simulink model "XFLUID02_reference"  (R2025a)
settings: Solver=ode23t  StartTime=0  StopTime=1.5  MaxStep=0.001  RelTol=1e-3  EnableMultiTasking=on
model workspace (MAT data in the model file):
  TRP_Par : object (value not decoded)
  fault_cylinder = 2
  inlet_area_factor = 1
  output_pressure_bar = 7
  pOutMeas_data = [7; 7]
  pOutMeas_time = [0; 1.5]
  pOut_Init_WKSP = 7
  pump_speed_rpm = 958
  seal_leak_fraction = 0
  speed_step_fraction = 0.08
  speed_step_time = 0.72
symbols that are objects in the model workspace (value not decoded): TRP_Par
undefined symbols (not defined in the file): Plunger, sm_pump_triplex_lib, smiData, X, Y, Z
libraries: sm_lib x133, fl_lib x62, nesl_utility x24, SimscapeFluids_lib x15, simulink x10, ee_lib x2
(part 2 of 7)

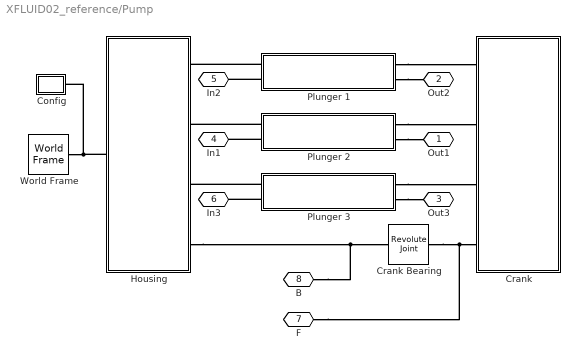
== system XFLUID02_reference/Pump ==
  Config : Subsystem
  Crank : Subsystem  mask(Crankshaft){shaft_len=shaft_len_P, shaft_rad=shaft_rad_P, web_rad=web_rad_P, web_len=web_len_P, motor_shaft_rad=motor_shaft_rad_P, motor_shaft_len=motor_shaft_len_P, shaft_pos=shaft_pos_P, crank_rho=crank_rho_P, motor_shaft_clr=motor_shaft_clr_P, crank_clr=crank_clr_P, crank_opc=crank_opc_P}
      mask prompts: shaft_pos "Crankpin Axis Offset (m)"; crank_rho "Density (kg/m^3)"; motor_shaft_clr "Motor Shaft Color [RGB]"; crank_clr "Crank Color [RGB]"; crank_opc "Opacity (0-1)"
      mask help: Models pump crankshaft with three crankpins, each offset by 120 degrees from the crankshaft axis.
      mask DialogControl text_radius Prompt: Radius (m)
      mask DialogControl text_length Prompt: Length (m)
      mask DialogControl text_crankpin Prompt: Crankpin
      mask DialogControl text_web Prompt: Web
      mask DialogControl text_motor_shaft Prompt: Motor Shaft
      mask DialogControl cont_crank_vis Prompt: Crankshaft Visualization
      mask Display: image('sm_pump_triplex_Crank_IMAGE.png');
  Crank Bearing : sm_lib/Joints/Revolute Joint  JointMode=Normal  CompositeWrenchDir=FollowerOnBase  CompositeWrenchFrame=BaseFrame  SenseConstraintForce=off  SenseConstraintTorque=off  SenseTotalForce=off  SenseTotalTorque=off  PositionTargetSpecify=off  PositionTargetPriority=High  PositionTargetValue=0  PositionTargetValueUnits=deg  VelocityTargetSpecify=off  VelocityTargetPriority=High  VelocityTargetValue=0  VelocityTargetValueUnits=deg/s  EquilibriumPosition=0  EquilibriumPositionUnits=deg  SpringStiffness=0  SpringStiffnessUnits=N*m/deg  DampingCoefficient=bearing_visc_frict  DampingCoefficientUnits=N*m/(deg/s)  LowerLimitSpecify=off  LowerLimitBound=-90  LowerLimitBoundUnits=deg  LowerLimitStiffness=1e4  LowerLimitStiffnessUnits=N*m/deg  LowerLimitDamping=10  LowerLimitDampingUnits=N*m/(deg/s)  LowerLimitTransitionRegionWidth=0.1  LowerLimitTransitionRegionWidthUnits=deg  UpperLimitSpecify=off  UpperLimitBound=90  UpperLimitBoundUnits=deg  UpperLimitStiffness=1e4  UpperLimitStiffnessUnits=N*m/deg  UpperLimitDamping=10  UpperLimitDampingUnits=N*m/(deg/s)  UpperLimitTransitionRegionWidth=0.1  UpperLimitTransitionRegionWidthUnits=deg  TorqueActuationMode=NoTorque  MotionActuationMode=ComputedMotion  SensePosition=off  SenseVelocity=off  SenseAcceleration=off  SenseTorqueForce=off  SenseLowerLimitTorqueForce=off  SenseUpperLimitTorqueForce=off
  Housing : Subsystem
      mask Display: image('sm_pump_triplex_Housing_IMAGE.png');
  Plunger 1 : Subsystem  AncestorBlock=sm_pump_triplex_lib/Plunger  mask(Hydraulic Plunger){cyl_gap=cyl_gap_P, cyl_rad_out=cyl_rad_out_P, cyl_len=cyl_len_P, cyl_stroke=cyl_stroke_P, cyl_rad_in=0, cyl_xc_rev=0, cyl_frict_brkway_frc=cyl_frict_brkway_frc_P, cyl_frict_brkway_vel=cyl_frict_brkway_vel_P, cyl_frict_col_frc=cyl_frict_col_frc_P, cyl_frict_visc_coef=cyl_frict_visc_coef_P, cyl_rho=cyl_rho_P, cyl_clr=cyl_clr_P, cyl_opc=cyl_opc_P, plgB_len=plgB_len_P, plgB_rad=plgB_rad_P, stem_len=stem_len_P, stem_rad=stem_rad_P, pin_len=pin_len_P, pin_rad=pin_rad_P, cup_rad_out=cup_rad_out_P, cup_thk=cup_thk_P, cup_len=cup_len_P, cup_pinOffset=cup_pinOffset_P, cup_rad_in=0, plg_rho=plg_rho_P, plg_clr=plg_clr_P, plg_opc=plg_opc_P, conrod_len=conrod_len_P, conrod_web_widP=conrod_web_widP_P, conrod_web_widC=conrod_web_widC_P, conrod_web_offC=0, conrod_web_offP=0, conrod_web_len=0, conrod_web_xc=0, conrod_ringC_wid=conrod_ringC_wid_P, conrod_ringP_wid=conrod_ringP_wid_P, crank_shaft_rad=crank_shaft_rad_P, conrod_ringC_or=0, conrod_ringP_or=0, conrod_ringC_xc_rev=0, conrod_ringP_xc_rev=0, conrod_thk=conrod_thk_P, conrod_rho=conrod_rho_P, conrod_clr=conrod_clr_P, conrod_opc=conrod_opc_P, chkv_in_maxA=chkv_in_maxA_P, chkv_out_maxA=chkv_out_maxA_P, chkv_press_set_popup=Set in Mask, chkv_in_crkP=chkv_in_crkP_P, chkv_out_crkP=chkv_out_crkP_P, chkv_in_maxOpenP=chkv_in_maxOpenP_P, chkv_out_maxOpenP=chkv_out_maxOpenP_P, chkv_vis_popup=Off, chkv_vis_rad_in=chkv_vis_rad_in_P, chkv_vis_rad_out=chkv_vis_rad_out_P, chkv_vis_clr_in=chkv_vis_clr_in_P, chkv_vis_clr_out=chkv_vis_clr_out_P, leak_cyl_popup=On, leak_cyl_area=1e-12+(fault_cylinder==1)*seal_leak_fraction*TRP_Par.Check_Valve.In.Max_Area, block_in_popup=On, block_in_factor=min(0.999,1-(fault_cylinder==1)*(1-inlet_area_factor)), seal_leak_vis_len=seal_leak_vis_len_P, seal_leak_vis_rad=seal_leak_vis_rad_P, seal_leak_vis_clr=seal_leak_vis_clr_P, seal_leak_vis_opc=0, inlet_obstr_len=inlet_obstr_len_P, inlet_obstr_rad=inlet_obstr_rad_P, inlet_obstr_xc_rev=0, inlet_obstr_clr=inlet_obstr_clr_P, inlet_obstr_opc=1}
      mask prompts: cyl_gap "Gap (m)"; cyl_rad_out "Outer radius (m)"; cyl_len "Length (m)"; cyl_stroke "Stroke (m)"; cyl_rad_in "Inner radius (m)"; cyl_xc_rev "Revolution Cross Section (m)"; cyl_frict_brkway_frc "Breakaway Friction Force (N)"; cyl_frict_brkway_vel "Breakaway Friction Velocity (m/s)"; cyl_frict_col_frc "Coulomb Friction Force (N)"; cyl_frict_visc_coef "Viscous Friction Coeff (N/(m/s))"; cyl_rho "Density (kg/m^3)"; cyl_clr "Color [RGB]"; cyl_opc "Opacity (0-1)"; cup_rad_out "Outer Radius (m)"; cup_thk "Wall Thickness (m)"; cup_len "Length(m)"; cup_pinOffset "Pin Offset (m)"; cup_rad_in "Inner Radius (m)"; plg_rho "Density (kg/m^3)"; plg_clr "Color [RGB]"; plg_opc "Opacity (0-1)"; conrod_len "Length, center-center (m)"; conrod_web_widP "Width, pin end (m)"; conrod_web_widC "Width, crank end (m)"; conrod_web_offC "Offset to shaft center (m)"; conrod_web_offP "Offset to pin center (m)"; conrod_web_len "Length web (m)"; conrod_web_xc "Extrusion cross section (m)"; conrod_ringC_wid "Crank Ring Width (m)"; conrod_ringP_wid "Pin Ring Width (m)"; crank_shaft_rad "Crank Shaft Radius (m)"; conrod_ringC_or "Outer Radius, Crank Ring"; conrod_ringP_or "Inner Radius, Pin Ring"; conrod_ringC_xc_rev "Crank Ring Cross Section (m)"; conrod_ringP_xc_rev "Pin Ring Cross Section (m)"; conrod_thk "Thickness (m)"; conrod_rho "Density (kg/m^3)"; conrod_clr "Color [RGB]"; conrod_opc "Opacity (0-1)"; chkv_press_set_popup "Pressure Settings"; chkv_vis_popup "Valve Visualization"; leak_cyl_popup "Seal Leak"; leak_cyl_area "Leak Area (m^2)"; block_in_popup "Blocked Inlet"; block_in_factor "Area Factor (0-1)"; seal_leak_vis_len "Length (m)"; seal_leak_vis_rad "Radius (m)"; seal_leak_vis_clr "Color [RGB]"; seal_leak_vis_opc "Opacity (0-1)"; inlet_obstr_len "Length (m)"; inlet_obstr_rad "Radius (m)"; inlet_obstr_xc_rev "Cross Section (m)"; inlet_obstr_clr "Color [RGB]"; inlet_obstr_opc "Opacity (0-1)"
      mask help: Models a single hydraulic plunger with hydraulic chamber. Two check valves control flow into and out of the hydraulic chamber. Degraded behavior can be modeled by enabling seal leakage and blocked inlet on the Faults tab. When "On, Run Time" is selected, MATLAB workspace variables set the parameters so that they can be tuned using Fast Restart.
      mask init:
      | % -- Configure submodels
      | % Fault: Seal Leak
      | if(leak_cyl_popup==1)
      |     set_param([gcb '/Seal Leak'],'OverrideUsingVariant','Off');
      |     seal_leak_vis_opc = 0;
      | elseif(leak_cyl_popup==2)
      |     set_param([gcb '/Seal Leak'],'OverrideUsingVariant','On');
      |     seal_leak_vis_opc = 1;
      | elseif(leak_cyl_popup==3)
      |     set_param([gcb '/Seal Leak'],'OverrideUsingVariant','Tune');
      |     seal_leak_vis_opc = 1;
      | end
      | 
      | % Fault: Blocked Inlet
      | inlet_obstr_xc_rev = [...
      |     inlet_obstr_rad                  -inlet_obstr_len/2;
      |     inlet_obstr_rad                   inlet_obstr_len/2;
      |     inlet_obstr_rad*block_in_factor   inlet_obstr_len/2;
      |     inlet_obstr_rad*block_in_factor  -inlet_obstr_len/2];
      | if(block_in_popup==1)
      |     set_param([gcb '/Check Valve Inlet'],...
      |         'area_max','chkv_in_maxA',...
      |         'area_max_conf','compiletime',...
      |         'BackgroundColor','[1 1 1]');
      |     inlet_obstr_opc = 0;
      | elseif(block_in_popup==2)
      |     set_param([gcb '/Check Valve Inlet'],...
      |         'area_max','chkv_in_maxA*block_in_factor',...
      |         'area_max_conf','compiletime',...
      |         'BackgroundColor','[1 0.9 0.9]');
      |     inlet_obstr_opc = 1;
      | elseif(block_in_popup==3)
      |     set_param([gcb '/Check Valve Inlet'],...
      |         'area_max','chkv_in_maxA_WKSP*block_in_factor_WKSP',...
      |         'area_max_conf','runtime',...
      |         'BackgroundColor','[1 0.9 0.9]');
      |     inlet_obstr_opc = 1;
      | end
      | 
      | % Parameter tuning: Check valve pressure settings
      | 
      | if(chkv_press_set_popup==1)
      |     set_param([gcb '/Check Valve Inlet'],...
      |         'p_crack_differential','chkv_in_crkP',...
      |         'p_crack_differential_conf','compiletime',...
      |         'press_max_differential','chkv_in_maxOpenP',...
      |         'press_max_differential_conf','compiletime');
      |     set_param([gcb '/Check Valve Outlet'],...
      |         'p_crack_differential','chkv_out_crkP',...
      |         'p_crack_differential_conf','compiletime',...
      |         'press_max_differential','chkv_out_maxOpenP',...
      |         'press_max_differential_conf','compiletime');
      | elseif(chkv_press_set_popup==2)
      |     set_param([gcb '/Check Valve Inlet'],...
      |         'p_crack_differential','chkv_all_crkP_WKSP',...
      |         'p_crack_differential_conf','runtime',...
      |         'press_max_differential','chkv_all_maxOpenP_WKSP',...
      |         'press_max_differential_conf','runtime');
      |     set_param([gcb '/Check Valve Outlet'],...
      |         'p_crack_differential','chkv_all_crkP_WKSP',...
      |         'p_crack_differential_conf','runtime',...
      |         'press_max_differential','chkv_all_maxOpenP_WKSP',...
      |         'press_max_differential_conf','runtime');
      | end
      | 
      | % Turn on/off visualization
      | if(chkv_vis_popup==1)
      |     set_param([gcb '/Valve Visual'],'OverrideUsingVariant','Off');
      | elseif(chkv_vis_popup==2)
      |     set_param([gcb '/Valve Visual'],'OverrideUsingVariant','On');
      | end
      | 
      | % -- Calculate derived parameters
      | % Cylinder: derived dimensions
      | cyl_rad_in  = plgB_rad + cyl_gap;
      | 
      | % Cylinder: cross-section for rev
      | cyl_xc_rev = [...
      |     cyl_rad_out  -cyl_len/2
      |     cyl_rad_out   cyl_len/2
      |     cyl_rad_in    cyl_len/2
      |     cyl_rad_in   -cyl_len/2];
      | 
      | % Stem Cup: cross-section for rev
      | cup_rad_in = cup_rad_out-cup_thk;
      | cup_xc_rev = [...
      |     cup_rad_out  -cup_len/2
      |     cup_rad_out   cup_len/2
      |     cup_rad_in    cup_len/2
      |     cup_rad_in   -cup_len/2];
      | 
      | % Connecting Rod, Crank Ring: cross-section for rev
      | conrod_ringC_or = crank_shaft_rad + conrod_ringC_wid;
      | conrod_ringC_xc_rev = [...
      |     conrod_ringC_or -conrod_thk/2*1.005;
      |     conrod_ringC_or  conrod_thk/2*1.005;
      |     crank_shaft_rad  conrod_thk/2*1.005;
      |     crank_shaft_rad -conrod_thk/2*1.005];
      | 
      | % Connecting Rod, Pin ring: cross-section for rev
      | conrod_ringP_or = pin_rad + conrod_ringP_wid;
      | conrod_ringP_xc_rev = [...
      |     conrod_ringP_or -conrod_thk/2*1.005;
      |     conrod_ringP_or  conrod_thk/2*1.005;
      |     pin_rad          conrod_thk/2*1.005;
      |     pin_rad         -conrod_thk/2*1.005];
      | 
      | % Connecting Rod, Web: cross-section for extrusion
      | conrod_web_offC = crank_shaft_rad + conrod_ringC_wid/2;
      | conrod_web_offP = pin_rad         + conrod_ringP_wid/2;
      | conrod_web_len  = conrod_len - conrod_web_offP - conrod_web_offC;
      | conrod_web_xc = [...
      |     -conrod_web_len -conrod_web_widC;
      |     conrod_web_len -conrod_web_widP;
      |     conrod_web_len  conrod_web_widP;
      |     -conrod_web_len  conrod_web_widC]/2;
      mask TypeOptions chkv_press_set_popup: Set in Mask | Tune at Run Time
      mask Callback chkv_press_set_popup:
      | maskObj = Simulink.Mask.get(gcb);
      | 
      | crPrP_h = maskObj.getDialogControl('text_open_crkP');
      | crMxP_h = maskObj.getDialogControl('text_open_maxOpenP');
      | crPIn_h = maskObj.getParameter('chkv_in_crkP');
      | crPOu_h = maskObj.getParameter('chkv_out_crkP');
      | mxPIn_h = maskObj.getParameter('chkv_in_maxOpenP');
      | mxPOu_h = maskObj.getParameter('chkv_out_maxOpenP');
      | 
      | allTxt_h = maskObj.getDialogControl('chkv_pres_set_all_tune_text');
      | 
      | temp_PressSetTune = get_param(gcb,'chkv_press_set_popup');
      | 
      | if (strcmp(temp_PressSetTune,'Set in Mask'))
      |     crPrP_h.Visible = 'on';
      |     crMxP_h.Visible = 'on';
      |     crPIn_h.Visible = 'on';
      |     crPOu_h.Visible = 'on';
      |     mxPIn_h.Visible = 'on';
      |     mxPOu_h.Visible = 'on';
      |     allTxt_h.Visible = 'off';
      |     outTxt_h.Visible = 'off';
      | else
      |     crPrP_h.Visible = 'off';
      |     crMxP_h.Visible = 'off';
      |     crPIn_h.Visible = 'off';
      |     crPOu_h.Visible = 'off';
      |     mxPIn_h.Visible = 'off';
      |     mxPOu_h.Visible = 'off';
      |     allTxt_h.Visible = 'on';
      |     outTxt_h.Visible = 'on';
      | end
      | clear maskObj temp_PressSetTune
      | clear crPrP_h crMxP_h crPIn_h crPOu_h mxPIn_h mxPOu_h
      | clear allTxt_h
      mask TypeOptions chkv_vis_popup: Off | On
      mask TypeOptions leak_cyl_popup: Off | On | On, Run Time
      mask Callback leak_cyl_popup:
      | maskObj = Simulink.Mask.get(gcb);
      | leak_area_h = maskObj.getParameter('leak_cyl_area');
      | leak_text_h = maskObj.getDialogControl('leak_cyl_tune_text');
      | if (strcmp(get_param(gcb,'leak_cyl_popup'),'Off'))
      |     leak_area_h.Visible = 'off';
      |     leak_text_h.Visible = 'off';
      | elseif (strcmp(get_param(gcb,'leak_cyl_popup'),'On'))
      |     leak_area_h.Visible = 'on';
      |     leak_text_h.Visible = 'off';
      | elseif (strcmp(get_param(gcb,'leak_cyl_popup'),'On, Run Time'))
      |     leak_area_h.Visible = 'off';
      |     leak_text_h.Visible = 'on';
      | end
      | %clear maskObj leak_area_h leak_text_h
      mask TypeOptions block_in_popup: Off | On | On, Run Time
      mask Callback block_in_popup:
      | maskObj = Simulink.Mask.get(gcb);
      | block_fctr_h = maskObj.getParameter('block_in_factor');
      | block_text_h = maskObj.getDialogControl('block_in_tune_text');
      | if (strcmp(get_param(gcb,'block_in_popup'),'Off'))
      |     block_fctr_h.Visible = 'off';
      |     block_text_h.Visible = 'off';
      | elseif (strcmp(get_param(gcb,'block_in_popup'),'On'))
      |     block_fctr_h.Visible = 'on';
      |     block_text_h.Visible = 'off';
      | elseif (strcmp(get_param(gcb,'block_in_popup'),'On, Run Time'))
      |     block_fctr_h.Visible = 'off';
      |     block_text_h.Visible = 'on';
      | end
      | clear maskObj block_fctr_h block_text_h
      mask DialogControl tab_cylinder Prompt: Cylinder
      mask DialogControl cont_dims Prompt: Dimensions
      mask DialogControl cont_friction Prompt: Friction
      mask DialogControl cont_cyl_vis Prompt: Cylinder Visualization
      mask DialogControl tab_plunger Prompt: Plunger
      mask DialogControl text_length Prompt: Length (m)
      mask DialogControl text_radius Prompt: Radius (m)
      mask DialogControl text_base Prompt: Base
      mask DialogControl text_stem Prompt: Stem
      mask DialogControl text_pin Prompt: Pin
      mask DialogControl cont_cup Prompt: Cup
      mask DialogControl cont_plg_vis Prompt: Plunger Visualization
      mask DialogControl tab_conrod Prompt: Rod
      mask DialogControl cont_conrodWeb Prompt: Web
      mask DialogControl cont_conrodRings Prompt: Rings
      mask DialogControl cont_conrod_vis Prompt: Rod Visualization
      mask DialogControl tab_valves Prompt: Valves
      mask DialogControl text_open_inlet Prompt: Inlet
      mask DialogControl text_open_outlet Prompt: Outlet
      mask DialogControl text_open_maxA Prompt: Max Area (m)
      mask DialogControl text_open_crkP Prompt: Crack. Pr (Pa)
      mask DialogControl text_open_maxOpenP Prompt: Max Pr. (Pa)
      mask DialogControl chkv_pres_set_all_tune_text Prompt: Set >> chkv_all_crkP_WKSP, chkv_all_maxOpenP_WKSP
      mask DialogControl cont_valve_vis Prompt: Visualization Settings
      mask DialogControl text_valvis_inlet Prompt: Inlet
      mask DialogControl text_valvis_out Prompt: Outlet
      mask DialogControl text_valvis_rad Prompt: Radius (m)
      mask DialogControl text_valvis_clr Prompt: Color [RGB]
      mask DialogControl tab_faults Prompt: Faults
      mask DialogControl leak_cyl_tune_text Prompt: Set >> leak_cyl_area_WKSP
      mask DialogControl block_in_tune_text Prompt: Set >> block_in_factor_WKSP, chkv_out_maxA_WKSP
      mask DialogControl cont_seal_leak_vis Prompt: Seal Leak Visualization
      mask DialogControl cont_blocked_line_vis Prompt: Blocked Line Visualization
      mask Display: image('sm_pump_triplex_Plunger_IMAGE.png');
  Plunger 2 : Subsystem  AncestorBlock=sm_pump_triplex_lib/Plunger  mask(Hydraulic Plunger){cyl_gap=cyl_gap_P, cyl_rad_out=cyl_rad_out_P, cyl_len=cyl_len_P, cyl_stroke=cyl_stroke_P, cyl_rad_in=0, cyl_xc_rev=0, cyl_frict_brkway_frc=cyl_frict_brkway_frc_P, cyl_frict_brkway_vel=cyl_frict_brkway_vel_P, cyl_frict_col_frc=cyl_frict_col_frc_P, cyl_frict_visc_coef=cyl_frict_visc_coef_P, cyl_rho=cyl_rho_P, cyl_clr=cyl_clr_P, cyl_opc=cyl_opc_P, plgB_len=plgB_len_P, plgB_rad=plgB_rad_P, stem_len=stem_len_P, stem_rad=stem_rad_P, pin_len=pin_len_P, pin_rad=pin_rad_P, cup_rad_out=cup_rad_out_P, cup_thk=cup_thk_P, cup_len=cup_len_P, cup_pinOffset=cup_pinOffset_P, cup_rad_in=0, plg_rho=plg_rho_P, plg_clr=plg_clr_P, plg_opc=plg_opc_P, conrod_len=conrod_len_P, conrod_web_widP=conrod_web_widP_P, conrod_web_widC=conrod_web_widC_P, conrod_web_offC=0, conrod_web_offP=0, conrod_web_len=0, conrod_web_xc=0, conrod_ringC_wid=conrod_ringC_wid_P, conrod_ringP_wid=conrod_ringP_wid_P, crank_shaft_rad=crank_shaft_rad_P, conrod_ringC_or=0, conrod_ringP_or=0, conrod_ringC_xc_rev=0, conrod_ringP_xc_rev=0, conrod_thk=conrod_thk_P, conrod_rho=conrod_rho_P, conrod_clr=conrod_clr_P, conrod_opc=conrod_opc_P, chkv_in_maxA=chkv_in_maxA_P, chkv_out_maxA=chkv_out_maxA_P, chkv_press_set_popup=Set in Mask, chkv_in_crkP=chkv_in_crkP_P, chkv_out_crkP=chkv_out_crkP_P, chkv_in_maxOpenP=chkv_in_maxOpenP_P, chkv_out_maxOpenP=chkv_out_maxOpenP_P, chkv_vis_popup=Off, chkv_vis_rad_in=chkv_vis_rad_in_P, chkv_vis_rad_out=chkv_vis_rad_out_P, chkv_vis_clr_in=chkv_vis_clr_in_P, chkv_vis_clr_out=chkv_vis_clr_out_P, leak_cyl_popup=On, leak_cyl_area=1e-12+(fault_cylinder==2)*seal_leak_fraction*TRP_Par.Check_Valve.In.Max_Area, block_in_popup=On, block_in_factor=min(0.999,1-(fault_cylinder==2)*(1-inlet_area_factor)), seal_leak_vis_len=seal_leak_vis_len_P, seal_leak_vis_rad=seal_leak_vis_rad_P, seal_leak_vis_clr=seal_leak_vis_clr_P, seal_leak_vis_opc=0, inlet_obstr_len=inlet_obstr_len_P, inlet_obstr_rad=inlet_obstr_rad_P, inlet_obstr_xc_rev=0, inlet_obstr_clr=inlet_obstr_clr_P, inlet_obstr_opc=1}
      mask prompts: cyl_gap "Gap (m)"; cyl_rad_out "Outer radius (m)"; cyl_len "Length (m)"; cyl_stroke "Stroke (m)"; cyl_rad_in "Inner radius (m)"; cyl_xc_rev "Revolution Cross Section (m)"; cyl_frict_brkway_frc "Breakaway Friction Force (N)"; cyl_frict_brkway_vel "Breakaway Friction Velocity (m/s)"; cyl_frict_col_frc "Coulomb Friction Force (N)"; cyl_frict_visc_coef "Viscous Friction Coeff (N/(m/s))"; cyl_rho "Density (kg/m^3)"; cyl_clr "Color [RGB]"; cyl_opc "Opacity (0-1)"; cup_rad_out "Outer Radius (m)"; cup_thk "Wall Thickness (m)"; cup_len "Length(m)"; cup_pinOffset "Pin Offset (m)"; cup_rad_in "Inner Radius (m)"; plg_rho "Density (kg/m^3)"; plg_clr "Color [RGB]"; plg_opc "Opacity (0-1)"; conrod_len "Length, center-center (m)"; conrod_web_widP "Width, pin end (m)"; conrod_web_widC "Width, crank end (m)"; conrod_web_offC "Offset to shaft center (m)"; conrod_web_offP "Offset to pin center (m)"; conrod_web_len "Length web (m)"; conrod_web_xc "Extrusion cross section (m)"; conrod_ringC_wid "Crank Ring Width (m)"; conrod_ringP_wid "Pin Ring Width (m)"; crank_shaft_rad "Crank Shaft Radius (m)"; conrod_ringC_or "Outer Radius, Crank Ring"; conrod_ringP_or "Inner Radius, Pin Ring"; conrod_ringC_xc_rev "Crank Ring Cross Section (m)"; conrod_ringP_xc_rev "Pin Ring Cross Section (m)"; conrod_thk "Thickness (m)"; conrod_rho "Density (kg/m^3)"; conrod_clr "Color [RGB]"; conrod_opc "Opacity (0-1)"; chkv_press_set_popup "Pressure Settings"; chkv_vis_popup "Valve Visualization"; leak_cyl_popup "Seal Leak"; leak_cyl_area "Leak Area (m^2)"; block_in_popup "Blocked Inlet"; block_in_factor "Area Factor (0-1)"; seal_leak_vis_len "Length (m)"; seal_leak_vis_rad "Radius (m)"; seal_leak_vis_clr "Color [RGB]"; seal_leak_vis_opc "Opacity (0-1)"; inlet_obstr_len "Length (m)"; inlet_obstr_rad "Radius (m)"; inlet_obstr_xc_rev "Cross Section (m)"; inlet_obstr_clr "Color [RGB]"; inlet_obstr_opc "Opacity (0-1)"
      mask help: Models a single hydraulic plunger with hydraulic chamber. Two check valves control flow into and out of the hydraulic chamber. Degraded behavior can be modeled by enabling seal leakage and blocked inlet on the Faults tab. When "On, Run Time" is selected, MATLAB workspace variables set the parameters so that they can be tuned using Fast Restart.
      mask init: same as XFLUID02_reference/Pump/Plunger 1
      mask TypeOptions chkv_press_set_popup: Set in Mask | Tune at Run Time
      mask Callback chkv_press_set_popup:
      | maskObj = Simulink.Mask.get(gcb);
      | 
      | crPrP_h = maskObj.getDialogControl('text_open_crkP');
      | crMxP_h = maskObj.getDialogControl('text_open_maxOpenP');
      | crPIn_h = maskObj.getParameter('chkv_in_crkP');
      | crPOu_h = maskObj.getParameter('chkv_out_crkP');
      | mxPIn_h = maskObj.getParameter('chkv_in_maxOpenP');
      | mxPOu_h = maskObj.getParameter('chkv_out_maxOpenP');
      | 
      | allTxt_h = maskObj.getDialogControl('chkv_pres_set_all_tune_text');
      | 
      | temp_PressSetTune = get_param(gcb,'chkv_press_set_popup');
      | 
      | if (strcmp(temp_PressSetTune,'Set in Mask'))
      |     crPrP_h.Visible = 'on';
      |     crMxP_h.Visible = 'on';
      |     crPIn_h.Visible = 'on';
      |     crPOu_h.Visible = 'on';
      |     mxPIn_h.Visible = 'on';
      |     mxPOu_h.Visible = 'on';
      |     allTxt_h.Visible = 'off';
      |     outTxt_h.Visible = 'off';
      | else
      |     crPrP_h.Visible = 'off';
      |     crMxP_h.Visible = 'off';
      |     crPIn_h.Visible = 'off';
      |     crPOu_h.Visible = 'off';
      |     mxPIn_h.Visible = 'off';
      |     mxPOu_h.Visible = 'off';
      |     allTxt_h.Visible = 'on';
      |     outTxt_h.Visible = 'on';
      | end
      | clear maskObj temp_PressSetTune
      | clear crPrP_h crMxP_h crPIn_h crPOu_h mxPIn_h mxPOu_h
      | clear allTxt_h
      mask TypeOptions chkv_vis_popup: Off | On
      mask TypeOptions leak_cyl_popup: Off | On | On, Run Time
      mask Callback leak_cyl_popup:
      | maskObj = Simulink.Mask.get(gcb);
      | leak_area_h = maskObj.getParameter('leak_cyl_area');
      | leak_text_h = maskObj.getDialogControl('leak_cyl_tune_text');
      | if (strcmp(get_param(gcb,'leak_cyl_popup'),'Off'))
      |     leak_area_h.Visible = 'off';
      |     leak_text_h.Visible = 'off';
      | elseif (strcmp(get_param(gcb,'leak_cyl_popup'),'On'))
      |     leak_area_h.Visible = 'on';
      |     leak_text_h.Visible = 'off';
      | elseif (strcmp(get_param(gcb,'leak_cyl_popup'),'On, Run Time'))
      |     leak_area_h.Visible = 'off';
      |     leak_text_h.Visible = 'on';
      | end
      | %clear maskObj leak_area_h leak_text_h
      mask TypeOptions block_in_popup: Off | On | On, Run Time
      mask Callback block_in_popup:
      | maskObj = Simulink.Mask.get(gcb);
      | block_fctr_h = maskObj.getParameter('block_in_factor');
      | block_text_h = maskObj.getDialogControl('block_in_tune_text');
      | if (strcmp(get_param(gcb,'block_in_popup'),'Off'))
      |     block_fctr_h.Visible = 'off';
      |     block_text_h.Visible = 'off';
      | elseif (strcmp(get_param(gcb,'block_in_popup'),'On'))
      |     block_fctr_h.Visible = 'on';
      |     block_text_h.Visible = 'off';
      | elseif (strcmp(get_param(gcb,'block_in_popup'),'On, Run Time'))
      |     block_fctr_h.Visible = 'off';
      |     block_text_h.Visible = 'on';
      | end
      | clear maskObj block_fctr_h block_text_h
      mask DialogControl tab_cylinder Prompt: Cylinder
      mask DialogControl cont_dims Prompt: Dimensions
      mask DialogControl cont_friction Prompt: Friction
      mask DialogControl cont_cyl_vis Prompt: Cylinder Visualization
      mask DialogControl tab_plunger Prompt: Plunger
      mask DialogControl text_length Prompt: Length (m)
      mask DialogControl text_radius Prompt: Radius (m)
      mask DialogControl text_base Prompt: Base
      mask DialogControl text_stem Prompt: Stem
      mask DialogControl text_pin Prompt: Pin
      mask DialogControl cont_cup Prompt: Cup
      mask DialogControl cont_plg_vis Prompt: Plunger Visualization
      mask DialogControl tab_conrod Prompt: Rod
      mask DialogControl cont_conrodWeb Prompt: Web
      mask DialogControl cont_conrodRings Prompt: Rings
      mask DialogControl cont_conrod_vis Prompt: Rod Visualization
      mask DialogControl tab_valves Prompt: Valves
      mask DialogControl text_open_inlet Prompt: Inlet
      mask DialogControl text_open_outlet Prompt: Outlet
      mask DialogControl text_open_maxA Prompt: Max Area (m)
      mask DialogControl text_open_crkP Prompt: Crack. Pr (Pa)
      mask DialogControl text_open_maxOpenP Prompt: Max Pr. (Pa)
      mask DialogControl chkv_pres_set_all_tune_text Prompt: Set >> chkv_all_crkP_WKSP, chkv_all_maxOpenP_WKSP
      mask DialogControl cont_valve_vis Prompt: Visualization Settings
      mask DialogControl text_valvis_inlet Prompt: Inlet
      mask DialogControl text_valvis_out Prompt: Outlet
      mask DialogControl text_valvis_rad Prompt: Radius (m)
      mask DialogControl text_valvis_clr Prompt: Color [RGB]
      mask DialogControl tab_faults Prompt: Faults
      mask DialogControl leak_cyl_tune_text Prompt: Set >> leak_cyl_area_WKSP
      mask DialogControl block_in_tune_text Prompt: Set >> block_in_factor_WKSP, chkv_out_maxA_WKSP
      mask DialogControl cont_seal_leak_vis Prompt: Seal Leak Visualization
      mask DialogControl cont_blocked_line_vis Prompt: Blocked Line Visualization
      mask Display: image('sm_pump_triplex_Plunger_IMAGE.png');
  Plunger 3 : Subsystem  AncestorBlock=sm_pump_triplex_lib/Plunger  mask(Hydraulic Plunger){cyl_gap=cyl_gap_P, cyl_rad_out=cyl_rad_out_P, cyl_len=cyl_len_P, cyl_stroke=cyl_stroke_P, cyl_rad_in=0, cyl_xc_rev=0, cyl_frict_brkway_frc=cyl_frict_brkway_frc_P, cyl_frict_brkway_vel=cyl_frict_brkway_vel_P, cyl_frict_col_frc=cyl_frict_col_frc_P, cyl_frict_visc_coef=cyl_frict_visc_coef_P, cyl_rho=cyl_rho_P, cyl_clr=cyl_clr_P, cyl_opc=cyl_opc_P, plgB_len=plgB_len_P, plgB_rad=plgB_rad_P, stem_len=stem_len_P, stem_rad=stem_rad_P, pin_len=pin_len_P, pin_rad=pin_rad_P, cup_rad_out=cup_rad_out_P, cup_thk=cup_thk_P, cup_len=cup_len_P, cup_pinOffset=cup_pinOffset_P, cup_rad_in=0, plg_rho=plg_rho_P, plg_clr=plg_clr_P, plg_opc=plg_opc_P, conrod_len=conrod_len_P, conrod_web_widP=conrod_web_widP_P, conrod_web_widC=conrod_web_widC_P, conrod_web_offC=0, conrod_web_offP=0, conrod_web_len=0, conrod_web_xc=0, conrod_ringC_wid=conrod_ringC_wid_P, conrod_ringP_wid=conrod_ringP_wid_P, crank_shaft_rad=crank_shaft_rad_P, conrod_ringC_or=0, conrod_ringP_or=0, conrod_ringC_xc_rev=0, conrod_ringP_xc_rev=0, conrod_thk=conrod_thk_P, conrod_rho=conrod_rho_P, conrod_clr=conrod_clr_P, conrod_opc=conrod_opc_P, chkv_in_maxA=chkv_in_maxA_P, chkv_out_maxA=chkv_out_maxA_P, chkv_press_set_popup=Set in Mask, chkv_in_crkP=chkv_in_crkP_P, chkv_out_crkP=chkv_out_crkP_P, chkv_in_maxOpenP=chkv_in_maxOpenP_P, chkv_out_maxOpenP=chkv_out_maxOpenP_P, chkv_vis_popup=Off, chkv_vis_rad_in=chkv_vis_rad_in_P, chkv_vis_rad_out=chkv_vis_rad_out_P, chkv_vis_clr_in=chkv_vis_clr_in_P, chkv_vis_clr_out=chkv_vis_clr_out_P, leak_cyl_popup=On, leak_cyl_area=1e-12+(fault_cylinder==3)*seal_leak_fraction*TRP_Par.Check_Valve.In.Max_Area, block_in_popup=On, block_in_factor=min(0.999,1-(fault_cylinder==3)*(1-inlet_area_factor)), seal_leak_vis_len=seal_leak_vis_len_P, seal_leak_vis_rad=seal_leak_vis_rad_P, seal_leak_vis_clr=seal_leak_vis_clr_P, seal_leak_vis_opc=0, inlet_obstr_len=inlet_obstr_len_P, inlet_obstr_rad=inlet_obstr_rad_P, inlet_obstr_xc_rev=0, inlet_obstr_clr=inlet_obstr_clr_P, inlet_obstr_opc=1}
      mask prompts: cyl_gap "Gap (m)"; cyl_rad_out "Outer radius (m)"; cyl_len "Length (m)"; cyl_stroke "Stroke (m)"; cyl_rad_in "Inner radius (m)"; cyl_xc_rev "Revolution Cross Section (m)"; cyl_frict_brkway_frc "Breakaway Friction Force (N)"; cyl_frict_brkway_vel "Breakaway Friction Velocity (m/s)"; cyl_frict_col_frc "Coulomb Friction Force (N)"; cyl_frict_visc_coef "Viscous Friction Coeff (N/(m/s))"; cyl_rho "Density (kg/m^3)"; cyl_clr "Color [RGB]"; cyl_opc "Opacity (0-1)"; cup_rad_out "Outer Radius (m)"; cup_thk "Wall Thickness (m)"; cup_len "Length(m)"; cup_pinOffset "Pin Offset (m)"; cup_rad_in "Inner Radius (m)"; plg_rho "Density (kg/m^3)"; plg_clr "Color [RGB]"; plg_opc "Opacity (0-1)"; conrod_len "Length, center-center (m)"; conrod_web_widP "Width, pin end (m)"; conrod_web_widC "Width, crank end (m)"; conrod_web_offC "Offset to shaft center (m)"; conrod_web_offP "Offset to pin center (m)"; conrod_web_len "Length web (m)"; conrod_web_xc "Extrusion cross section (m)"; conrod_ringC_wid "Crank Ring Width (m)"; conrod_ringP_wid "Pin Ring Width (m)"; crank_shaft_rad "Crank Shaft Radius (m)"; conrod_ringC_or "Outer Radius, Crank Ring"; conrod_ringP_or "Inner Radius, Pin Ring"; conrod_ringC_xc_rev "Crank Ring Cross Section (m)"; conrod_ringP_xc_rev "Pin Ring Cross Section (m)"; conrod_thk "Thickness (m)"; conrod_rho "Density (kg/m^3)"; conrod_clr "Color [RGB]"; conrod_opc "Opacity (0-1)"; chkv_press_set_popup "Pressure Settings"; chkv_vis_popup "Valve Visualization"; leak_cyl_popup "Seal Leak"; leak_cyl_area "Leak Area (m^2)"; block_in_popup "Blocked Inlet"; block_in_factor "Area Factor (0-1)"; seal_leak_vis_len "Length (m)"; seal_leak_vis_rad "Radius (m)"; seal_leak_vis_clr "Color [RGB]"; seal_leak_vis_opc "Opacity (0-1)"; inlet_obstr_len "Length (m)"; inlet_obstr_rad "Radius (m)"; inlet_obstr_xc_rev "Cross Section (m)"; inlet_obstr_clr "Color [RGB]"; inlet_obstr_opc "Opacity (0-1)"
      mask help: Models a single hydraulic plunger with hydraulic chamber. Two check valves control flow into and out of the hydraulic chamber. Degraded behavior can be modeled by enabling seal leakage and blocked inlet on the Faults tab. When "On, Run Time" is selected, MATLAB workspace variables set the parameters so that they can be tuned using Fast Restart.
      mask init: same as XFLUID02_reference/Pump/Plunger 1
      mask TypeOptions chkv_press_set_popup: Set in Mask | Tune at Run Time
      mask Callback chkv_press_set_popup:
      | maskObj = Simulink.Mask.get(gcb);
      | 
      | crPrP_h = maskObj.getDialogControl('text_open_crkP');
      | crMxP_h = maskObj.getDialogControl('text_open_maxOpenP');
      | crPIn_h = maskObj.getParameter('chkv_in_crkP');
      | crPOu_h = maskObj.getParameter('chkv_out_crkP');
      | mxPIn_h = maskObj.getParameter('chkv_in_maxOpenP');
      | mxPOu_h = maskObj.getParameter('chkv_out_maxOpenP');
      | 
      | allTxt_h = maskObj.getDialogControl('chkv_pres_set_all_tune_text');
      | 
      | temp_PressSetTune = get_param(gcb,'chkv_press_set_popup');
      | 
      | if (strcmp(temp_PressSetTune,'Set in Mask'))
      |     crPrP_h.Visible = 'on';
      |     crMxP_h.Visible = 'on';
      |     crPIn_h.Visible = 'on';
      |     crPOu_h.Visible = 'on';
      |     mxPIn_h.Visible = 'on';
      |     mxPOu_h.Visible = 'on';
      |     allTxt_h.Visible = 'off';
      |     outTxt_h.Visible = 'off';
      | else
      |     crPrP_h.Visible = 'off';
      |     crMxP_h.Visible = 'off';
      |     crPIn_h.Visible = 'off';
      |     crPOu_h.Visible = 'off';
      |     mxPIn_h.Visible = 'off';
      |     mxPOu_h.Visible = 'off';
      |     allTxt_h.Visible = 'on';
      |     outTxt_h.Visible = 'on';
      | end
      | clear maskObj temp_PressSetTune
      | clear crPrP_h crMxP_h crPIn_h crPOu_h mxPIn_h mxPOu_h
      | clear allTxt_h
      mask TypeOptions chkv_vis_popup: Off | On
      mask TypeOptions leak_cyl_popup: Off | On | On, Run Time
      mask Callback leak_cyl_popup:
      | maskObj = Simulink.Mask.get(gcb);
      | leak_area_h = maskObj.getParameter('leak_cyl_area');
      | leak_text_h = maskObj.getDialogControl('leak_cyl_tune_text');
      | if (strcmp(get_param(gcb,'leak_cyl_popup'),'Off'))
      |     leak_area_h.Visible = 'off';
      |     leak_text_h.Visible = 'off';
      | elseif (strcmp(get_param(gcb,'leak_cyl_popup'),'On'))
      |     leak_area_h.Visible = 'on';
      |     leak_text_h.Visible = 'off';
      | elseif (strcmp(get_param(gcb,'leak_cyl_popup'),'On, Run Time'))
      |     leak_area_h.Visible = 'off';
      |     leak_text_h.Visible = 'on';
      | end
      | %clear maskObj leak_area_h leak_text_h
      mask TypeOptions block_in_popup: Off | On | On, Run Time
      mask Callback block_in_popup:
      | maskObj = Simulink.Mask.get(gcb);
      | block_fctr_h = maskObj.getParameter('block_in_factor');
      | block_text_h = maskObj.getDialogControl('block_in_tune_text');
      | if (strcmp(get_param(gcb,'block_in_popup'),'Off'))
      |     block_fctr_h.Visible = 'off';
      |     block_text_h.Visible = 'off';
      | elseif (strcmp(get_param(gcb,'block_in_popup'),'On'))
      |     block_fctr_h.Visible = 'on';
      |     block_text_h.Visible = 'off';
      | elseif (strcmp(get_param(gcb,'block_in_popup'),'On, Run Time'))
      |     block_fctr_h.Visible = 'off';
      |     block_text_h.Visible = 'on';
      | end
      | clear maskObj block_fctr_h block_text_h
      mask DialogControl tab_cylinder Prompt: Cylinder
      mask DialogControl cont_dims Prompt: Dimensions
      mask DialogControl cont_friction Prompt: Friction
      mask DialogControl cont_cyl_vis Prompt: Cylinder Visualization
      mask DialogControl tab_plunger Prompt: Plunger
      mask DialogControl text_length Prompt: Length (m)
      mask DialogControl text_radius Prompt: Radius (m)
      mask DialogControl text_base Prompt: Base
      mask DialogControl text_stem Prompt: Stem
      mask DialogControl text_pin Prompt: Pin
      mask DialogControl cont_cup Prompt: Cup
      mask DialogControl cont_plg_vis Prompt: Plunger Visualization
      mask DialogControl tab_conrod Prompt: Rod
      mask DialogControl cont_conrodWeb Prompt: Web
      mask DialogControl cont_conrodRings Prompt: Rings
      mask DialogControl cont_conrod_vis Prompt: Rod Visualization
      mask DialogControl tab_valves Prompt: Valves
      mask DialogControl text_open_inlet Prompt: Inlet
      mask DialogControl text_open_outlet Prompt: Outlet
      mask DialogControl text_open_maxA Prompt: Max Area (m)
      mask DialogControl text_open_crkP Prompt: Crack. Pr (Pa)
      mask DialogControl text_open_maxOpenP Prompt: Max Pr. (Pa)
      mask DialogControl chkv_pres_set_all_tune_text Prompt: Set >> chkv_all_crkP_WKSP, chkv_all_maxOpenP_WKSP
      mask DialogControl cont_valve_vis Prompt: Visualization Settings
      mask DialogControl text_valvis_inlet Prompt: Inlet
      mask DialogControl text_valvis_out Prompt: Outlet
      mask DialogControl text_valvis_rad Prompt: Radius (m)
      mask DialogControl text_valvis_clr Prompt: Color [RGB]
      mask DialogControl tab_faults Prompt: Faults
      mask DialogControl leak_cyl_tune_text Prompt: Set >> leak_cyl_area_WKSP
      mask DialogControl block_in_tune_text Prompt: Set >> block_in_factor_WKSP, chkv_out_maxA_WKSP
      mask DialogControl cont_seal_leak_vis Prompt: Seal Leak Visualization
      mask DialogControl cont_blocked_line_vis Prompt: Blocked Line Visualization
      mask Display: image('sm_pump_triplex_Plunger_IMAGE.png');
  World Frame : sm_lib/Frames and Transforms/World Frame
  Out1 : PMIOPort  Side=Right
  Out2 : PMIOPort  Port=2  Side=Right
  Out3 : PMIOPort  Port=3  Side=Right
  In1 : PMIOPort  Port=4  Side=Right
  In2 : PMIOPort  Port=5  Side=Right
  In3 : PMIOPort  Port=6  Side=Right
  F : PMIOPort  Port=7  Side=Left
  B : PMIOPort  Port=8  Side=Left
  connections:
  Housing/LConn1 -- World Frame/RConn1 -- Config/RConn1
  Plunger 2/LConn1 -- Housing/RConn2
  Plunger 1/LConn2 -- In2/RConn1
  Plunger 1/RConn1 -- Crank/LConn1
  Plunger 2/RConn1 -- Crank/LConn2
  Plunger 3/LConn2 -- In3/RConn1
  Plunger 3/RConn2 -- Out3/RConn1
  Plunger 1/LConn1 -- Housing/RConn1
  Plunger 2/LConn2 -- In1/RConn1
  Plunger 3/LConn1 -- Housing/RConn3
  Housing/RConn4 -- B/RConn1 -- Crank Bearing/LConn1
  Crank Bearing/RConn1 -- F/RConn1 -- Crank/LConn4
  Plunger 1/RConn2 -- Out2/RConn1
  Plunger 2/RConn2 -- Out1/RConn1
  Plunger 3/RConn1 -- Crank/LConn3

== system XFLUID02_reference/Sensing Current ==
  Current Sensor : fl_lib/Electrical/Electrical Sensors/Current Sensor
  Current with Noise : Scope  NumInputPorts=2
      settings: ActiveDisplayYMinimum=-5.56656  ActiveDisplayYMaximum=49.76256  DataLoggingVariableName=ScopeData2
  Measurement Noise : simulink/Sources/Band-Limited White Noise  Cov=TRP_Par.Sensors.i.Np  Ts=TRP_Par.Sensors.i.Ts  seed=[23345]
  PS-Simulink Converter : nesl_utility/PS-Simulink Converter  PhysicalDomain=network_engine_domain  SubClassName=ps_output  LeftPortType=input  RightPortType=output  PseudoPeriodic=off  Frequencies=[]  VectorFormat=1-D array  Unit=1  AffineConversion=off
  Sum1 : Sum  Inputs=++|
  Zero-Order Hold : ZeroOrderHold  SampleTime=TRP_Par.Sensors.i.Ts
  - : PMIOPort  Side=Right
  + : PMIOPort  Port=2  Side=Left
  wires:
  Measurement Noise/1 -> Sum1/1  "Noise"
  Sum1/1 -> Zero-Order Hold/1
  PS-Simulink Converter/1 -> Sum1/2, Current with Noise/2
  Zero-Order Hold/1 -> Current with Noise/1
  connections:
  PS-Simulink Converter/LConn1 -- Current Sensor/RConn1
  +/RConn1 -- Current Sensor/LConn1
  Current Sensor/RConn2 -- -/RConn1

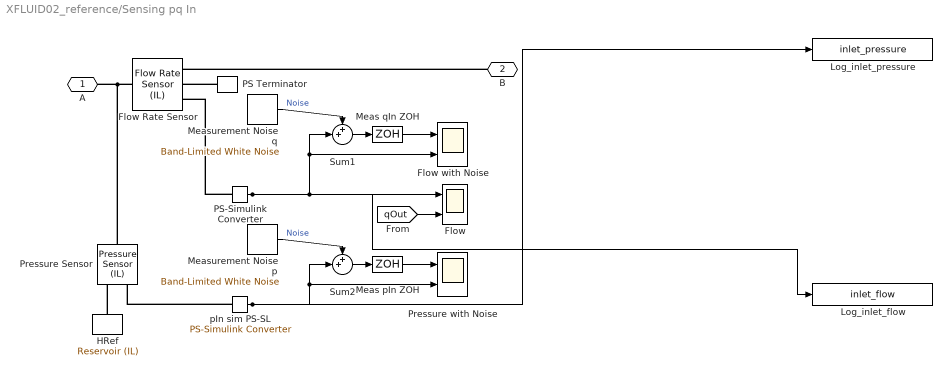
== system XFLUID02_reference/Sensing pq In ==
  Flow : Scope  NumInputPorts=2
      settings: ActiveDisplayYMinimum=-6.56594  ActiveDisplayYMaximum=59.09339  DataLoggingVariableName=ScopeData2
  Flow Rate Sensor : fl_lib/Isothermal Liquid/Sensors/Flow Rate Sensor (IL)  sensor_type=3
      settings: InternalSimscapePortConfiguration="{\"Bottom\":[],\"Left\":[{\"id\":\"A\",\"label\":\"A\",\"type\":\"foundation.isothermal_liquid.isothermal_liquid\"}],\"Right\":[{\"id\":\"B\",\"label\":\"B\",\"type\":\"foundation.isothermal_liquid.isothermal_liquid\"},{\"id\":\"M\",\"label\":\"M\",\"type\":\"output\"},{\"id\":\"V\",\"label\":\"V\",\"type\":\"output\"}],\"Top\":[]}"
      settings: LibrarySourceBlock=|
      | fl_lib/Hydraulic/Hydraulic Sensors/Hydraulic Flow Rate
      | Sensor
  Flow with Noise : Scope  NumInputPorts=2
      settings: ActiveDisplayYMinimum=-7.18648  ActiveDisplayYMaximum=60.19336
  HRef : fl_lib/Isothermal Liquid/Elements/Reservoir (IL)  reservoir_type=foundation.enum.constant_controlled.constant  pressure_spec=foundation.enum.pressure_spec.atmospheric  reservoir_pressure=0.101325 MPa
      settings: LibrarySourceBlock=fl_lib/Hydraulic/Hydraulic Elements/Hydraulic Reference
  Log_inlet_flow : ToWorkspace  VariableName=inlet_flow  SaveFormat=Timeseries  SampleTime=-1
  Log_inlet_pressure : ToWorkspace  VariableName=inlet_pressure  SaveFormat=Timeseries  SampleTime=-1
  Meas pIn ZOH : ZeroOrderHold  SampleTime=TRP_Par.Sensors.p.Ts
  Meas qIn ZOH : ZeroOrderHold  SampleTime=TRP_Par.Sensors.q.Ts
  Measurement Noise p : simulink/Sources/Band-Limited White Noise  Cov=TRP_Par.Sensors.p.Np  Ts=TRP_Par.Sensors.p.Ts  seed=[23345]
  Measurement Noise q : simulink/Sources/Band-Limited White Noise  Cov=TRP_Par.Sensors.q.Np  Ts=TRP_Par.Sensors.q.Ts  seed=[23345]
  PS Terminator : fl_lib/Physical Signals/Sinks/PS Terminator
  PS-Simulink Converter : nesl_utility/PS-Simulink Converter  PhysicalDomain=network_engine_domain  SubClassName=ps_output  LeftPortType=input  RightPortType=output  PseudoPeriodic=off  Frequencies=[]  VectorFormat=1-D array  Unit=lpm  AffineConversion=off
  Pressure Sensor : fl_lib/Isothermal Liquid/Sensors/Pressure Sensor (IL)  pressure_measure=foundation.enum.pressure_measure.difference
      settings: InternalSimscapePortConfiguration="{\"Bottom\":[],\"Left\":[{\"id\":\"A\",\"label\":\"A\",\"type\":\"foundation.isothermal_liquid.isothermal_liquid\"}],\"Right\":[{\"id\":\"B\",\"label\":\"B\",\"type\":\"foundation.isothermal_liquid.isothermal_liquid\"},{\"id\":\"P\",\"label\":\"P\",\"type\":\"output\"}],\"Top\":[]}"
      settings: LibrarySourceBlock=|
      | fl_lib/Hydraulic/Hydraulic Sensors/Hydraulic Pressure
      | Sensor
  Pressure with Noise : Scope  NumInputPorts=2
      settings: ActiveDisplayYMinimum=6.95483  ActiveDisplayYMaximum=7.36166
  Sum1 : Sum  Inputs=++|
  Sum2 : Sum  Inputs=++|
  pIn sim PS-SL : nesl_utility/PS-Simulink Converter  PhysicalDomain=network_engine_domain  SubClassName=ps_output  LeftPortType=input  RightPortType=output  PseudoPeriodic=off  Frequencies=[]  VectorFormat=1-D array  Unit=bar  AffineConversion=off
  A : PMIOPort  Side=Left
  B : PMIOPort  Port=2  Side=Right
  wires:
  Meas pIn ZOH/1 -> Pressure with Noise/1
  Measurement Noise p/1 -> Sum2/1  "Noise"
  pIn sim PS-SL/1 -> Pressure with Noise/2, Sum2/2, Log_inlet_pressure/1
  Sum2/1 -> Meas pIn ZOH/1
  Meas qIn ZOH/1 -> Flow with Noise/1
  Sum1/1 -> Meas qIn ZOH/1
  Measurement Noise q/1 -> Sum1/1  "Noise"
  PS-Simulink Converter/1 -> Flow/1, Flow with Noise/2, Sum1/2, Log_inlet_flow/1
  [qOut] -> Flow/2
  connections:
  pIn sim PS-SL/LConn1 -- Pressure Sensor/RConn2
  HRef/LConn1 -- Pressure Sensor/RConn1
  Pressure Sensor/LConn1 -- Flow Rate Sensor/LConn1 -- A/RConn1
  PS Terminator/LConn1 -- Flow Rate Sensor/RConn2
  B/RConn1 -- Flow Rate Sensor/RConn1
  PS-Simulink Converter/LConn1 -- Flow Rate Sensor/RConn3

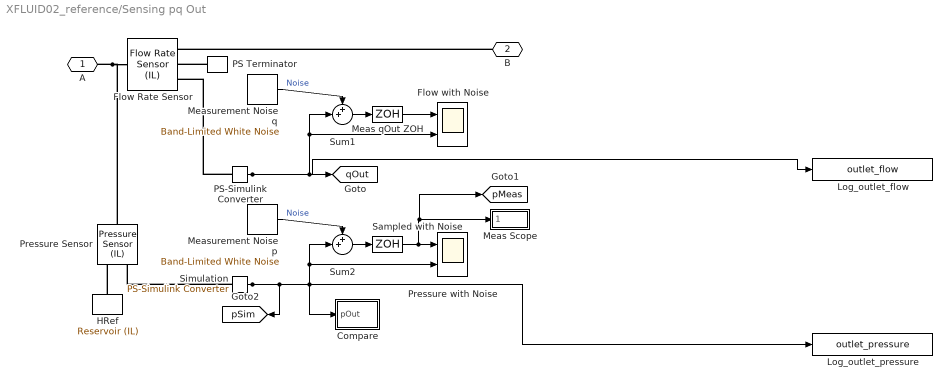
== system XFLUID02_reference/Sensing pq Out ==
  Compare : Subsystem
  Flow Rate Sensor : fl_lib/Isothermal Liquid/Sensors/Flow Rate Sensor (IL)  sensor_type=3
      settings: InternalSimscapePortConfiguration="{\"Bottom\":[],\"Left\":[{\"id\":\"A\",\"label\":\"A\",\"type\":\"foundation.isothermal_liquid.isothermal_liquid\"}],\"Right\":[{\"id\":\"B\",\"label\":\"B\",\"type\":\"foundation.isothermal_liquid.isothermal_liquid\"},{\"id\":\"M\",\"label\":\"M\",\"type\":\"output\"},{\"id\":\"V\",\"label\":\"V\",\"type\":\"output\"}],\"Top\":[]}"
      settings: LibrarySourceBlock=|
      | fl_lib/Hydraulic/Hydraulic Sensors/Hydraulic Flow Rate
      | Sensor
  Flow with Noise : Scope  NumInputPorts=2
      settings: ActiveDisplayYMinimum=-6.25341  ActiveDisplayYMaximum=51.79569
  HRef : fl_lib/Isothermal Liquid/Elements/Reservoir (IL)  reservoir_type=foundation.enum.constant_controlled.constant  pressure_spec=foundation.enum.pressure_spec.atmospheric  reservoir_pressure=0.101325 MPa
      settings: LibrarySourceBlock=fl_lib/Hydraulic/Hydraulic Elements/Hydraulic Reference
  Log_outlet_flow : ToWorkspace  VariableName=outlet_flow  SaveFormat=Timeseries  SampleTime=-1
  Log_outlet_pressure : ToWorkspace  VariableName=outlet_pressure  SaveFormat=Timeseries  SampleTime=-1
  Meas Scope : Subsystem
  Meas qOut ZOH : ZeroOrderHold  SampleTime=TRP_Par.Sensors.q.Ts
  Measurement Noise p : simulink/Sources/Band-Limited White Noise  Cov=TRP_Par.Sensors.p.Np  Ts=TRP_Par.Sensors.p.Ts  seed=[23345]
  Measurement Noise q : simulink/Sources/Band-Limited White Noise  Cov=TRP_Par.Sensors.q.Np  Ts=TRP_Par.Sensors.q.Ts  seed=[23345]
  PS Terminator : fl_lib/Physical Signals/Sinks/PS Terminator
  PS-Simulink Converter : nesl_utility/PS-Simulink Converter  PhysicalDomain=network_engine_domain  SubClassName=ps_output  LeftPortType=input  RightPortType=output  PseudoPeriodic=off  Frequencies=[]  VectorFormat=1-D array  Unit=lpm  AffineConversion=off
  Pressure Sensor : fl_lib/Isothermal Liquid/Sensors/Pressure Sensor (IL)  pressure_measure=foundation.enum.pressure_measure.difference
      settings: InternalSimscapePortConfiguration="{\"Bottom\":[],\"Left\":[{\"id\":\"A\",\"label\":\"A\",\"type\":\"foundation.isothermal_liquid.isothermal_liquid\"}],\"Right\":[{\"id\":\"B\",\"label\":\"B\",\"type\":\"foundation.isothermal_liquid.isothermal_liquid\"},{\"id\":\"P\",\"label\":\"P\",\"type\":\"output\"}],\"Top\":[]}"
      settings: LibrarySourceBlock=|
      | fl_lib/Hydraulic/Hydraulic Sensors/Hydraulic Pressure
      | Sensor
  Pressure with Noise : Scope  NumInputPorts=2
      settings: ActiveDisplayYMinimum=6.95483  ActiveDisplayYMaximum=7.36166
  Sampled with Noise : ZeroOrderHold  SampleTime=TRP_Par.Sensors.p.Ts
  Simulation : nesl_utility/PS-Simulink Converter  PhysicalDomain=network_engine_domain  SubClassName=ps_output  LeftPortType=input  RightPortType=output  PseudoPeriodic=off  Frequencies=[]  VectorFormat=1-D array  Unit=bar  AffineConversion=off
  Sum1 : Sum  Inputs=++|
  Sum2 : Sum  Inputs=++|
  A : PMIOPort  Side=Left
  B : PMIOPort  Port=2  Side=Right
  tag scope: pMeas=global, pSim=global, qOut=global
  wires:
  PS-Simulink Converter/1 -> Sum1/2, Flow with Noise/2, [qOut], Log_outlet_flow/1
  Measurement Noise q/1 -> Sum1/1  "Noise"
  Sum1/1 -> Meas qOut ZOH/1
  Meas qOut ZOH/1 -> Flow with Noise/1
  Sum2/1 -> Sampled with Noise/1
  Simulation/1 -> [pSim], Compare/1(pOut), Sum2/2, Pressure with Noise/2, Log_outlet_pressure/1
  Measurement Noise p/1 -> Sum2/1  "Noise"
  Sampled with Noise/1 -> [pMeas], Meas Scope/1(pMeas), Pressure with Noise/1
  connections:
  Pressure Sensor/LConn1 -- Flow Rate Sensor/LConn1 -- A/RConn1
  HRef/LConn1 -- Pressure Sensor/RConn1
  Simulation/LConn1 -- Pressure Sensor/RConn2
  PS Terminator/LConn1 -- Flow Rate Sensor/RConn2
  B/RConn1 -- Flow Rate Sensor/RConn1
  PS-Simulink Converter/LConn1 -- Flow Rate Sensor/RConn3

== system XFLUID02_reference/Diagnostics/Diagnostics ==
  "pOut " : Inport
  Off : Subsystem  VariantControl=Off
  On : Subsystem  VariantControl=On
  " fault" : Outport  VectorParamsAs1DForOutWhenUnconnected=off
  " hmi" : Outport  Port=2  VectorParamsAs1DForOutWhenUnconnected=off

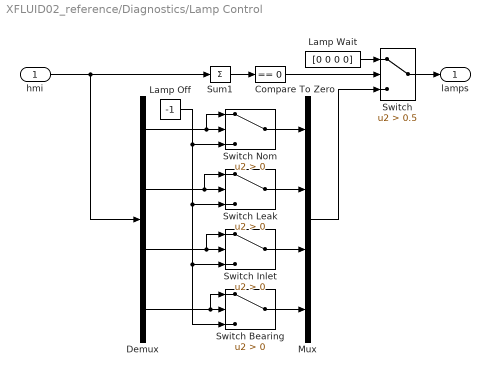
== system XFLUID02_reference/Diagnostics/Lamp Control ==
  hmi : Inport
  Compare To Zero : simulink/Logic and Bit Operations/Compare To Zero  relop===  OutDataTypeStr=boolean  ZeroCross=off
  Demux : Demux
  Lamp Off : Constant  Value=-1
  Lamp Wait : Constant  Value=[0 0 0 0]
  Mux : Mux
  Sum1 : Sum  Inputs=+
  Switch : Switch  Criteria=u2 > Threshold  Threshold=0.5  ZeroCross=off  SaturateOnIntegerOverflow=off  InputSameDT=off
  Switch Bearing : Switch  Criteria=u2 > Threshold  ZeroCross=off  SaturateOnIntegerOverflow=off  InputSameDT=off
  Switch Inlet : Switch  Criteria=u2 > Threshold  ZeroCross=off  SaturateOnIntegerOverflow=off  InputSameDT=off
  Switch Leak : Switch  Criteria=u2 > Threshold  ZeroCross=off  SaturateOnIntegerOverflow=off  InputSameDT=off
  Switch Nom : Switch  Criteria=u2 > Threshold  ZeroCross=off  SaturateOnIntegerOverflow=off  InputSameDT=off
  lamps : Outport  VectorParamsAs1DForOutWhenUnconnected=off
  wires:
  Compare To Zero/1 -> Switch/2
  Sum1/1 -> Compare To Zero/1
  hmi/1 -> Demux/1, Sum1/1
  Switch/1 -> lamps/1
  Lamp Wait/1 -> Switch/1
  Switch Nom/1 -> Mux/1
  Switch Leak/1 -> Mux/2
  Switch Inlet/1 -> Mux/3
  Switch Bearing/1 -> Mux/4
  Mux/1 -> Switch/3
  Demux/1 -> Switch Nom/1, Switch Nom/2
  Demux/2 -> Switch Leak/1, Switch Leak/2
  Demux/3 -> Switch Inlet/1, Switch Inlet/2
  Demux/4 -> Switch Bearing/1, Switch Bearing/2
  Lamp Off/1 -> Switch Bearing/3, Switch Inlet/3, Switch Leak/3, Switch Nom/3

== system XFLUID02_reference/Driver/Driver ==
  Dyno : Subsystem  VariantControl=Dyno
      mask Display: image('sm_pump_triplex_driverDyno_IMAGE.png');
  Motor : Subsystem  VariantControl=Motor  mask{winding_fault_enable=Off, winding_fault_sw=0}
      mask prompts: winding_fault_enable "Winding Fault"; winding_fault_sw "Winding Fault Input for Switch (1,2)"
      mask init:
      | if(strcmp(get_param(gcb,'winding_fault_enable'),'Off'))
      |     winding_fault_sw = 1;
      | else
      |     winding_fault_sw = 2;
      | end
      mask TypeOptions winding_fault_enable: Off | On
      mask Display:
      | image('sm_pump_triplex_driverMotor_IMAGE.png');
      | 
      | color('red');
      | if(strcmp(get_param(gcb,'winding_fault_enable'),'On'))
      |     plot([0.85 0.6],[1.1 0.9])
      |     plot([0.6 0.85],[1.1 0.9])
      | end
      | 
      | % Plot points to set plot range
      | color('white');plot(1.2,2.4);plot(-1.2,-2.4)
      | color('black');
  " F " : PMIOPort  Side=Right
  " B " : PMIOPort  Port=2  Side=Right
  " + " : PMIOPort  Port=3  Side=Left
  " - " : PMIOPort  Port=4  Side=Left
